simulink model "phase_mixer_simulink"  (R2024b)
settings: Solver=ode45  StartTime=0.0  StopTime=2e-9  FixedStep=4e-13  MaxStep=4e-13  RelTol=1e-3
undefined symbols (not defined in the file or in its folder): tau
settings Model: Creator=Menna  LastModifiedBy=Menna

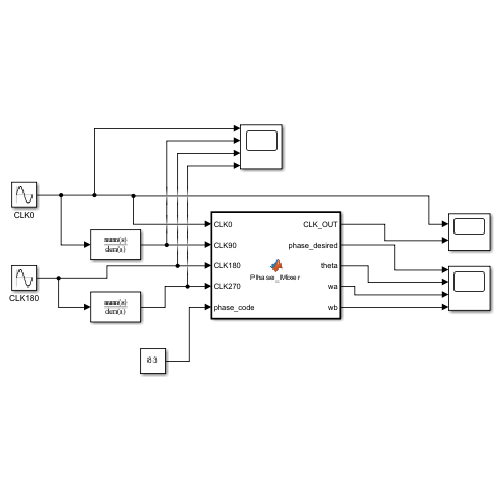
[thumbnail: Simulink's stored preview of the top-level diagram]
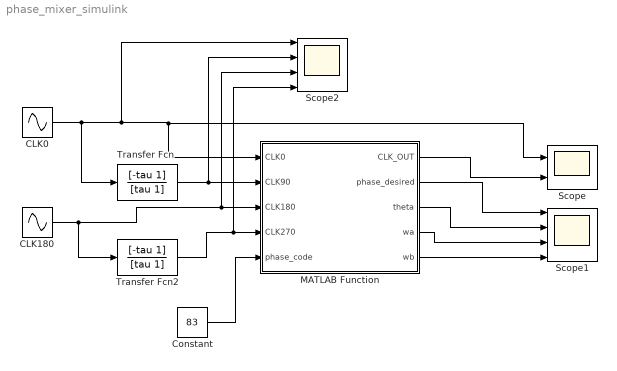
== system phase_mixer_simulink ==
  CLK0 : Sin  Frequency=2*pi*2.5e9  Phase=pi/2  SampleTime=0
  CLK180 : Sin  Frequency=2*pi*2.5e9  Phase=-pi/2  SampleTime=0
  Constant : Constant  Value=83  OutDataTypeStr=uint8
  MATLAB Function : MATLAB Function  TreatAsAtomicUnit=on
  Scope : Scope  NumInputPorts=2
  Scope1 : Scope  NumInputPorts=4
  Scope2 : Scope  NumInputPorts=4
  Transfer Fcn : TransferFcn  Numerator=[-tau 1]  Denominator=[tau 1]
  Transfer Fcn2 : TransferFcn  Numerator=[-tau 1]  Denominator=[tau 1]
  wires:
  CLK0/1 -> Transfer Fcn/1, Scope2/1, Scope/1, MATLAB Function/1(CLK0)
  CLK180/1 -> Transfer Fcn2/1, Scope2/3, MATLAB Function/3(CLK180)
  Constant/1 -> MATLAB Function/5(phase_code)
  MATLAB Function/2(phase_desired) -> Scope1/1
  MATLAB Function/3(theta) -> Scope1/2
  MATLAB Function/4(wa) -> Scope1/3
  MATLAB Function/5(wb) -> Scope1/4
  MATLAB Function/1(CLK_OUT) -> Scope/2
  Transfer Fcn/1 -> Scope2/2, MATLAB Function/2(CLK90)
  Transfer Fcn2/1 -> Scope2/4, MATLAB Function/4(CLK270)

== matlab function phase_mixer_simulink/MATLAB Function ==
  data: CLK0 input; CLK_OUT output; CLK90 input; CLK180 input; CLK270 input; phase_code input; phase_desired output; theta output; wa output; wb output
function [CLK_OUT, phase_desired, theta, wa, wb] = ...
    Phase_Mixer(CLK0, CLK90, CLK180, CLK270, phase_code)

%% Decode the 8-bits
binary = dec2bin(phase_code,8);
phase_quadrant = binary(1:2);   % First 2 bits
phase_angle = binary(3:8);  % Remaining 6 bits
decimal_quad = bin2dec(phase_quadrant);
decimal_angle = bin2dec(phase_angle);

%% calculate theta

theta = (90/64)*decimal_angle;

%% Quadrant Selection

switch decimal_quad

    case 0
        CLK_A = CLK0;
        CLK_B = CLK90;

    case 1
        CLK_A = CLK90;
        CLK_B = CLK180;

    case 2
        CLK_A = CLK180;
        CLK_B = CLK270;

    otherwise
        CLK_A = CLK270;
        CLK_B = CLK0;

end

%% wa and wb

wa = cos(theta*(pi/180));
wb = sin(theta*(pi/180)); %rana

%% output clock 

CLK_OUT = wa * CLK_A + wb * CLK_B;


%% phase comparison

phase_desired = decimal_quad*90 + theta;

end
